simulink model "fft_direct_maptail_test"  (Simulink 7.2)
settings: Solver=VariableStepDiscrete  StartTime=0.0  StopTime=250  RelTol=1e-3
libraries: xbsIndex_r4 x1029, casper_library_misc x88, simulink x2
(part 6 of 9)

== system fft_direct_maptail_test/fft_direct/butterfly1_1/twiddle ==
  a : Inport
  b : Inport  Port=2
  sync : Inport  Port=3
  AddSub : xbsIndex_r4/AddSub  mode=Subtraction  use_carryin=off  use_carryout=off  en=off  latency=add_latency  precision=Full  arith_type=Unsigned  n_bits=16  bin_pt=14  quantization=Truncate  overflow=Wrap  dbl_ovrd=off  use_behavioral_HDL=on  hw_selection=Fabric  pipelined=off  block_type=addsub
  AddSub1 : xbsIndex_r4/AddSub  mode=Addition  use_carryin=off  use_carryout=off  en=off  latency=add_latency  precision=Full  arith_type=Unsigned  n_bits=16  bin_pt=14  quantization=Truncate  overflow=Wrap  dbl_ovrd=off  use_behavioral_HDL=on  hw_selection=Fabric  pipelined=off  block_type=addsub
  c_to_ri1 : casper_library_misc/c_to_ri  SystemSampleTime=-1  n_bits=input_bit_width  bin_pt=input_bit_width-1
      settings: AttributesFormatString=16_15 r/i
  c_to_ri2 : casper_library_misc/c_to_ri  SystemSampleTime=-1  n_bits=coeff_bit_width  bin_pt=coeff_bit_width-2
      settings: AttributesFormatString=16_14 r/i
  c_to_ri3 : casper_library_misc/c_to_ri  SystemSampleTime=-1  n_bits=input_bit_width  bin_pt=input_bit_width-1
      settings: AttributesFormatString=16_15 r/i
  coeff_gen : Subsystem  AncestorBlock=casper_library_ffts_twiddle_coeff_gen/coeff_gen  mask(coeff_gen){Coeffs=getfield( getfield( get_param( gcb,'UserData' ), 'parameters'),'Coeffs'), coeff_bit_width=16, StepPeriod=0, bram_latency=2, coeffs_bram=off}
      mask prompts: Coeffs "Coefficients: (0 to 2^(FFTSize-1)-1)"; coeff_bit_width "Coefficient Bit Width:"; StepPeriod "Step Period: (2^?)"; bram_latency "Latency:"; coeffs_bram "Store coefficients in BRAM"
      mask help: Generates a sequence of complex coefficients
      mask init:
      | coeff_gen_init( gcb, ...
      |     'Coeffs', Coeffs, ...
      |     'coeff_bit_width', coeff_bit_width, ...
      |     'StepPeriod', StepPeriod, ...
      |     'bram_latency', bram_latency, ...
      |     'coeffs_bram', coeffs_bram);
      settings: AttributesFormatString=4 @ (16,14)
      mask CallbackString:
      | Coeffs = eval(get_param(gcb, 'Coeffs'));
      | if( length(Coeffs) == 1 ),
      |     set_param(gcb, 'MaskVisibilities',{'on','on','off','off','off'});
      | else
      |     set_param(gcb, 'MaskVisibilities',{'on','on','on','on','on'});
      | end||||
  convert0 : xbsIndex_r4/Convert  arith_type="Signed  (2's comp)"  n_bits=input_bit_width+4  bin_pt=input_bit_width+1  quantization=Truncate  overflow=Wrap  latency=conv_latency  dbl_ovrd=off  pipeline=on  block_type=convert
      settings: block_version=11.4
  convert1 : xbsIndex_r4/Convert  arith_type="Signed  (2's comp)"  n_bits=input_bit_width+4  bin_pt=input_bit_width+1  quantization=Truncate  overflow=Wrap  latency=conv_latency  dbl_ovrd=off  pipeline=on  block_type=convert
      settings: block_version=11.4
  delay0 : xbsIndex_r4/Delay  en=off  latency=mult_latency + add_latency + bram_latency + conv_latency  dbl_ovrd=off  reg_retiming=off  block_type=delay
      settings: block_version=11.4
  delay1 : xbsIndex_r4/Delay  en=off  latency=bram_latency  dbl_ovrd=off  reg_retiming=on  block_type=delay
      settings: block_version=11.4
  delay2 : xbsIndex_r4/Delay  en=off  latency=mult_latency + add_latency + bram_latency + conv_latency  dbl_ovrd=off  reg_retiming=off  block_type=delay
      settings: block_version=11.4
  mult{,1..3} (4 alike) : xbsIndex_r4/Mult  precision=Full  arith_type="Signed  (2's comp)"  n_bits=16  bin_pt=14  quantization=Truncate  overflow=Wrap  en=off  latency=mult_latency  dbl_ovrd=off  use_behavioral_HDL=on  opt=Speed  use_embedded=off  optimum_pipeline=off  pipeline=on  use_rpm=on  placement_style=Triangular  block_type=mult
      settings: block_version=11.4
  a_re : Outport
  a_im : Outport  Port=2
  bw_re : Outport  Port=3
  bw_im : Outport  Port=4
  sync_out : Outport  Port=5
  wires:
  a/1 -> delay0/1
  delay0/1 -> c_to_ri1/1
  c_to_ri1/1 -> a_re/1
  c_to_ri1/2 -> a_im/1
  sync/1 -> delay2/1, coeff_gen/1(rst)
  delay2/1 -> sync_out/1
  coeff_gen/1(w) -> c_to_ri2/1
  b/1 -> delay1/1
  delay1/1 -> c_to_ri3/1
  c_to_ri3/1 -> mult/1, mult3/1
  c_to_ri2/1 -> mult/2, mult1/2
  c_to_ri3/2 -> mult1/1, mult2/1
  c_to_ri2/2 -> mult2/2, mult3/2
  mult/1 -> AddSub/1
  mult1/1 -> AddSub1/1
  mult2/1 -> AddSub/2
  mult3/1 -> AddSub1/2
  AddSub/1 -> convert0/1
  convert0/1 -> bw_re/1
  AddSub1/1 -> convert1/1
  convert1/1 -> bw_im/1

== system fft_direct_maptail_test/fft_direct/butterfly1_2/convert_of1 ==
  din : Inport  OutDataType=sfix(16)  OutScaling=2^0
  all_0s : xbsIndex_r4/Logical  logical_function=NAND  inputs=4  en=off  latency=latency  precision=Full  arith_type=Unsigned  n_bits=16  bin_pt=0  align_bp=on  dbl_ovrd=off  block_type=logical
  all_1s : xbsIndex_r4/Logical  logical_function=NAND  inputs=4  en=off  latency=latency  precision=Full  arith_type=Unsigned  n_bits=16  bin_pt=0  align_bp=on  dbl_ovrd=off  block_type=logical
  and : xbsIndex_r4/Logical  logical_function=AND  inputs=2  en=off  latency=0  precision=Full  arith_type=Unsigned  n_bits=16  bin_pt=0  align_bp=on  dbl_ovrd=off  block_type=logical
  convert : xbsIndex_r4/Convert  arith_type="Signed  (2's comp)"  n_bits=bit_width_o  bin_pt=binary_point_o  quantization=Truncate  overflow=Wrap  latency=latency  dbl_ovrd=off  pipeline=on  block_type=convert
      settings: block_version=10.1.1
  invert{1..4} (4 alike) : xbsIndex_r4/Inverter  en=off  latency=0  dbl_ovrd=off  block_type=inv
      invert3 settings: block_version=11.4
      invert4 settings: block_version=11.4
  slice1 : xbsIndex_r4/Slice  nbits=1  boolean_output=on  mode=Upper Bit Location + Width  bit1=0  base1=MSB of Input  bit0=0  base0=LSB of Input  dbl_ovrd=off  block_type=slice
      settings: infoedit="Extracts a given range of bits from each input sample and presents it at the output.  The output type is ordinarily unsigned with binary point at zero, but can be Boolean when the slice is one bit wide.<P><P>Hardware notes: In hardware this block costs nothing."  block_version=10.1.1
  slice2 : xbsIndex_r4/Slice  nbits=1  boolean_output=on  mode=Upper Bit Location + Width  bit1=-1  base1=MSB of Input  bit0=0  base0=LSB of Input  dbl_ovrd=off  block_type=slice
      settings: infoedit="Extracts a given range of bits from each input sample and presents it at the output.  The output type is ordinarily unsigned with binary point at zero, but can be Boolean when the slice is one bit wide.<P><P>Hardware notes: In hardware this block costs nothing."  block_version=10.1.1
  slice3 : xbsIndex_r4/Slice  nbits=1  boolean_output=on  mode=Upper Bit Location + Width  bit1=-2  base1=MSB of Input  bit0=0  base0=LSB of Input  dbl_ovrd=off  block_type=slice
  slice4 : xbsIndex_r4/Slice  nbits=1  boolean_output=on  mode=Upper Bit Location + Width  bit1=-3  base1=MSB of Input  bit0=0  base0=LSB of Input  dbl_ovrd=off  block_type=slice
  dout : Outport
  of : Outport  Port=2
  wires:
  din/1 -> convert/1, slice1/1, slice2/1, slice3/1, slice4/1
  convert/1 -> dout/1
  slice1/1 -> all_1s/1, invert1/1
  invert1/1 -> all_0s/1
  slice2/1 -> all_1s/2, invert2/1
  invert2/1 -> all_0s/2
  slice3/1 -> all_1s/3, invert3/1
  invert3/1 -> all_0s/3
  slice4/1 -> all_1s/4, invert4/1
  invert4/1 -> all_0s/4
  all_0s/1 -> and/1
  all_1s/1 -> and/2
  and/1 -> of/1

== system fft_direct_maptail_test/fft_direct/butterfly1_2/convert_of2 ==
  din : Inport  OutDataType=sfix(16)  OutScaling=2^0
  all_0s : xbsIndex_r4/Logical  logical_function=NAND  inputs=4  en=off  latency=latency  precision=Full  arith_type=Unsigned  n_bits=16  bin_pt=0  align_bp=on  dbl_ovrd=off  block_type=logical
  all_1s : xbsIndex_r4/Logical  logical_function=NAND  inputs=4  en=off  latency=latency  precision=Full  arith_type=Unsigned  n_bits=16  bin_pt=0  align_bp=on  dbl_ovrd=off  block_type=logical
  and : xbsIndex_r4/Logical  logical_function=AND  inputs=2  en=off  latency=0  precision=Full  arith_type=Unsigned  n_bits=16  bin_pt=0  align_bp=on  dbl_ovrd=off  block_type=logical
  convert : xbsIndex_r4/Convert  arith_type="Signed  (2's comp)"  n_bits=bit_width_o  bin_pt=binary_point_o  quantization=Truncate  overflow=Wrap  latency=latency  dbl_ovrd=off  pipeline=on  block_type=convert
      settings: block_version=10.1.1
  invert{1..4} (4 alike) : xbsIndex_r4/Inverter  en=off  latency=0  dbl_ovrd=off  block_type=inv
      invert3 settings: block_version=11.4
      invert4 settings: block_version=11.4
  slice1 : xbsIndex_r4/Slice  nbits=1  boolean_output=on  mode=Upper Bit Location + Width  bit1=0  base1=MSB of Input  bit0=0  base0=LSB of Input  dbl_ovrd=off  block_type=slice
      settings: infoedit="Extracts a given range of bits from each input sample and presents it at the output.  The output type is ordinarily unsigned with binary point at zero, but can be Boolean when the slice is one bit wide.<P><P>Hardware notes: In hardware this block costs nothing."  block_version=10.1.1
  slice2 : xbsIndex_r4/Slice  nbits=1  boolean_output=on  mode=Upper Bit Location + Width  bit1=-1  base1=MSB of Input  bit0=0  base0=LSB of Input  dbl_ovrd=off  block_type=slice
      settings: infoedit="Extracts a given range of bits from each input sample and presents it at the output.  The output type is ordinarily unsigned with binary point at zero, but can be Boolean when the slice is one bit wide.<P><P>Hardware notes: In hardware this block costs nothing."  block_version=10.1.1
  slice3 : xbsIndex_r4/Slice  nbits=1  boolean_output=on  mode=Upper Bit Location + Width  bit1=-2  base1=MSB of Input  bit0=0  base0=LSB of Input  dbl_ovrd=off  block_type=slice
  slice4 : xbsIndex_r4/Slice  nbits=1  boolean_output=on  mode=Upper Bit Location + Width  bit1=-3  base1=MSB of Input  bit0=0  base0=LSB of Input  dbl_ovrd=off  block_type=slice
  dout : Outport
  of : Outport  Port=2
  wires:
  din/1 -> convert/1, slice1/1, slice2/1, slice3/1, slice4/1
  convert/1 -> dout/1
  slice1/1 -> all_1s/1, invert1/1
  invert1/1 -> all_0s/1
  slice2/1 -> all_1s/2, invert2/1
  invert2/1 -> all_0s/2
  slice3/1 -> all_1s/3, invert3/1
  invert3/1 -> all_0s/3
  slice4/1 -> all_1s/4, invert4/1
  invert4/1 -> all_0s/4
  all_0s/1 -> and/1
  all_1s/1 -> and/2
  and/1 -> of/1

== system fft_direct_maptail_test/fft_direct/butterfly1_2/convert_of3 ==
  din : Inport  OutDataType=sfix(16)  OutScaling=2^0
  all_0s : xbsIndex_r4/Logical  logical_function=NAND  inputs=4  en=off  latency=latency  precision=Full  arith_type=Unsigned  n_bits=16  bin_pt=0  align_bp=on  dbl_ovrd=off  block_type=logical
  all_1s : xbsIndex_r4/Logical  logical_function=NAND  inputs=4  en=off  latency=latency  precision=Full  arith_type=Unsigned  n_bits=16  bin_pt=0  align_bp=on  dbl_ovrd=off  block_type=logical
  and : xbsIndex_r4/Logical  logical_function=AND  inputs=2  en=off  latency=0  precision=Full  arith_type=Unsigned  n_bits=16  bin_pt=0  align_bp=on  dbl_ovrd=off  block_type=logical
  convert : xbsIndex_r4/Convert  arith_type="Signed  (2's comp)"  n_bits=bit_width_o  bin_pt=binary_point_o  quantization=Truncate  overflow=Wrap  latency=latency  dbl_ovrd=off  pipeline=on  block_type=convert
      settings: block_version=10.1.1
  invert{1..4} (4 alike) : xbsIndex_r4/Inverter  en=off  latency=0  dbl_ovrd=off  block_type=inv
      invert3 settings: block_version=11.4
      invert4 settings: block_version=11.4
  slice1 : xbsIndex_r4/Slice  nbits=1  boolean_output=on  mode=Upper Bit Location + Width  bit1=0  base1=MSB of Input  bit0=0  base0=LSB of Input  dbl_ovrd=off  block_type=slice
      settings: infoedit="Extracts a given range of bits from each input sample and presents it at the output.  The output type is ordinarily unsigned with binary point at zero, but can be Boolean when the slice is one bit wide.<P><P>Hardware notes: In hardware this block costs nothing."  block_version=10.1.1
  slice2 : xbsIndex_r4/Slice  nbits=1  boolean_output=on  mode=Upper Bit Location + Width  bit1=-1  base1=MSB of Input  bit0=0  base0=LSB of Input  dbl_ovrd=off  block_type=slice
      settings: infoedit="Extracts a given range of bits from each input sample and presents it at the output.  The output type is ordinarily unsigned with binary point at zero, but can be Boolean when the slice is one bit wide.<P><P>Hardware notes: In hardware this block costs nothing."  block_version=10.1.1
  slice3 : xbsIndex_r4/Slice  nbits=1  boolean_output=on  mode=Upper Bit Location + Width  bit1=-2  base1=MSB of Input  bit0=0  base0=LSB of Input  dbl_ovrd=off  block_type=slice
  slice4 : xbsIndex_r4/Slice  nbits=1  boolean_output=on  mode=Upper Bit Location + Width  bit1=-3  base1=MSB of Input  bit0=0  base0=LSB of Input  dbl_ovrd=off  block_type=slice
  dout : Outport
  of : Outport  Port=2
  wires:
  din/1 -> convert/1, slice1/1, slice2/1, slice3/1, slice4/1
  convert/1 -> dout/1
  slice1/1 -> all_1s/1, invert1/1
  invert1/1 -> all_0s/1
  slice2/1 -> all_1s/2, invert2/1
  invert2/1 -> all_0s/2
  slice3/1 -> all_1s/3, invert3/1
  invert3/1 -> all_0s/3
  slice4/1 -> all_1s/4, invert4/1
  invert4/1 -> all_0s/4
  all_0s/1 -> and/1
  all_1s/1 -> and/2
  and/1 -> of/1

== system fft_direct_maptail_test/fft_direct/butterfly1_2/convert_of4 ==
  din : Inport  OutDataType=sfix(16)  OutScaling=2^0
  all_0s : xbsIndex_r4/Logical  logical_function=NAND  inputs=4  en=off  latency=latency  precision=Full  arith_type=Unsigned  n_bits=16  bin_pt=0  align_bp=on  dbl_ovrd=off  block_type=logical
  all_1s : xbsIndex_r4/Logical  logical_function=NAND  inputs=4  en=off  latency=latency  precision=Full  arith_type=Unsigned  n_bits=16  bin_pt=0  align_bp=on  dbl_ovrd=off  block_type=logical
  and : xbsIndex_r4/Logical  logical_function=AND  inputs=2  en=off  latency=0  precision=Full  arith_type=Unsigned  n_bits=16  bin_pt=0  align_bp=on  dbl_ovrd=off  block_type=logical
  convert : xbsIndex_r4/Convert  arith_type="Signed  (2's comp)"  n_bits=bit_width_o  bin_pt=binary_point_o  quantization=Truncate  overflow=Wrap  latency=latency  dbl_ovrd=off  pipeline=on  block_type=convert
      settings: block_version=10.1.1
  invert{1..4} (4 alike) : xbsIndex_r4/Inverter  en=off  latency=0  dbl_ovrd=off  block_type=inv
      invert3 settings: block_version=11.4
      invert4 settings: block_version=11.4
  slice1 : xbsIndex_r4/Slice  nbits=1  boolean_output=on  mode=Upper Bit Location + Width  bit1=0  base1=MSB of Input  bit0=0  base0=LSB of Input  dbl_ovrd=off  block_type=slice
      settings: infoedit="Extracts a given range of bits from each input sample and presents it at the output.  The output type is ordinarily unsigned with binary point at zero, but can be Boolean when the slice is one bit wide.<P><P>Hardware notes: In hardware this block costs nothing."  block_version=10.1.1
  slice2 : xbsIndex_r4/Slice  nbits=1  boolean_output=on  mode=Upper Bit Location + Width  bit1=-1  base1=MSB of Input  bit0=0  base0=LSB of Input  dbl_ovrd=off  block_type=slice
      settings: infoedit="Extracts a given range of bits from each input sample and presents it at the output.  The output type is ordinarily unsigned with binary point at zero, but can be Boolean when the slice is one bit wide.<P><P>Hardware notes: In hardware this block costs nothing."  block_version=10.1.1
  slice3 : xbsIndex_r4/Slice  nbits=1  boolean_output=on  mode=Upper Bit Location + Width  bit1=-2  base1=MSB of Input  bit0=0  base0=LSB of Input  dbl_ovrd=off  block_type=slice
  slice4 : xbsIndex_r4/Slice  nbits=1  boolean_output=on  mode=Upper Bit Location + Width  bit1=-3  base1=MSB of Input  bit0=0  base0=LSB of Input  dbl_ovrd=off  block_type=slice
  dout : Outport
  of : Outport  Port=2
  wires:
  din/1 -> convert/1, slice1/1, slice2/1, slice3/1, slice4/1
  convert/1 -> dout/1
  slice1/1 -> all_1s/1, invert1/1
  invert1/1 -> all_0s/1
  slice2/1 -> all_1s/2, invert2/1
  invert2/1 -> all_0s/2
  slice3/1 -> all_1s/3, invert3/1
  invert3/1 -> all_0s/3
  slice4/1 -> all_1s/4, invert4/1
  invert4/1 -> all_0s/4
  all_0s/1 -> and/1
  all_1s/1 -> and/2
  and/1 -> of/1

== system fft_direct_maptail_test/fft_direct/butterfly1_2/twiddle ==
  a : Inport
  b : Inport  Port=2
  sync : Inport  Port=3
  AddSub : xbsIndex_r4/AddSub  mode=Subtraction  use_carryin=off  use_carryout=off  en=off  latency=add_latency  precision=Full  arith_type=Unsigned  n_bits=16  bin_pt=14  quantization=Truncate  overflow=Wrap  dbl_ovrd=off  use_behavioral_HDL=on  hw_selection=Fabric  pipelined=off  block_type=addsub
  AddSub1 : xbsIndex_r4/AddSub  mode=Addition  use_carryin=off  use_carryout=off  en=off  latency=add_latency  precision=Full  arith_type=Unsigned  n_bits=16  bin_pt=14  quantization=Truncate  overflow=Wrap  dbl_ovrd=off  use_behavioral_HDL=on  hw_selection=Fabric  pipelined=off  block_type=addsub
  c_to_ri1 : casper_library_misc/c_to_ri  SystemSampleTime=-1  n_bits=input_bit_width  bin_pt=input_bit_width-1
      settings: AttributesFormatString=16_15 r/i
  c_to_ri2 : casper_library_misc/c_to_ri  SystemSampleTime=-1  n_bits=coeff_bit_width  bin_pt=coeff_bit_width-2
      settings: AttributesFormatString=16_14 r/i
  c_to_ri3 : casper_library_misc/c_to_ri  SystemSampleTime=-1  n_bits=input_bit_width  bin_pt=input_bit_width-1
      settings: AttributesFormatString=16_15 r/i
  coeff_gen : Subsystem  AncestorBlock=casper_library_ffts_twiddle_coeff_gen/coeff_gen  mask(coeff_gen){Coeffs=getfield( getfield( get_param( gcb,'UserData' ), 'parameters'),'Coeffs'), coeff_bit_width=16, StepPeriod=0, bram_latency=2, coeffs_bram=off}
      mask prompts: Coeffs "Coefficients: (0 to 2^(FFTSize-1)-1)"; coeff_bit_width "Coefficient Bit Width:"; StepPeriod "Step Period: (2^?)"; bram_latency "Latency:"; coeffs_bram "Store coefficients in BRAM"
      mask help: Generates a sequence of complex coefficients
      mask init:
      | coeff_gen_init( gcb, ...
      |     'Coeffs', Coeffs, ...
      |     'coeff_bit_width', coeff_bit_width, ...
      |     'StepPeriod', StepPeriod, ...
      |     'bram_latency', bram_latency, ...
      |     'coeffs_bram', coeffs_bram);
      settings: AttributesFormatString=4 @ (16,14)
      mask CallbackString:
      | Coeffs = eval(get_param(gcb, 'Coeffs'));
      | if( length(Coeffs) == 1 ),
      |     set_param(gcb, 'MaskVisibilities',{'on','on','off','off','off'});
      | else
      |     set_param(gcb, 'MaskVisibilities',{'on','on','on','on','on'});
      | end||||
  convert0 : xbsIndex_r4/Convert  arith_type="Signed  (2's comp)"  n_bits=input_bit_width+4  bin_pt=input_bit_width+1  quantization=Truncate  overflow=Wrap  latency=conv_latency  dbl_ovrd=off  pipeline=on  block_type=convert
      settings: block_version=11.4
  convert1 : xbsIndex_r4/Convert  arith_type="Signed  (2's comp)"  n_bits=input_bit_width+4  bin_pt=input_bit_width+1  quantization=Truncate  overflow=Wrap  latency=conv_latency  dbl_ovrd=off  pipeline=on  block_type=convert
      settings: block_version=11.4
  delay0 : xbsIndex_r4/Delay  en=off  latency=mult_latency + add_latency + bram_latency + conv_latency  dbl_ovrd=off  reg_retiming=off  block_type=delay
      settings: block_version=11.4
  delay1 : xbsIndex_r4/Delay  en=off  latency=bram_latency  dbl_ovrd=off  reg_retiming=on  block_type=delay
      settings: block_version=11.4
  delay2 : xbsIndex_r4/Delay  en=off  latency=mult_latency + add_latency + bram_latency + conv_latency  dbl_ovrd=off  reg_retiming=off  block_type=delay
      settings: block_version=11.4
  mult{,1..3} (4 alike) : xbsIndex_r4/Mult  precision=Full  arith_type="Signed  (2's comp)"  n_bits=16  bin_pt=14  quantization=Truncate  overflow=Wrap  en=off  latency=mult_latency  dbl_ovrd=off  use_behavioral_HDL=on  opt=Speed  use_embedded=off  optimum_pipeline=off  pipeline=on  use_rpm=on  placement_style=Triangular  block_type=mult
      settings: block_version=11.4
  a_re : Outport
  a_im : Outport  Port=2
  bw_re : Outport  Port=3
  bw_im : Outport  Port=4
  sync_out : Outport  Port=5
  wires:
  a/1 -> delay0/1
  delay0/1 -> c_to_ri1/1
  c_to_ri1/1 -> a_re/1
  c_to_ri1/2 -> a_im/1
  sync/1 -> delay2/1, coeff_gen/1(rst)
  delay2/1 -> sync_out/1
  coeff_gen/1(w) -> c_to_ri2/1
  b/1 -> delay1/1
  delay1/1 -> c_to_ri3/1
  c_to_ri3/1 -> mult/1, mult3/1
  c_to_ri2/1 -> mult/2, mult1/2
  c_to_ri3/2 -> mult1/1, mult2/1
  c_to_ri2/2 -> mult2/2, mult3/2
  mult/1 -> AddSub/1
  mult1/1 -> AddSub1/1
  mult2/1 -> AddSub/2
  mult3/1 -> AddSub1/2
  AddSub/1 -> convert0/1
  convert0/1 -> bw_re/1
  AddSub1/1 -> convert1/1
  convert1/1 -> bw_im/1

== system fft_direct_maptail_test/fft_direct/butterfly1_3/convert_of1 ==
  din : Inport  OutDataType=sfix(16)  OutScaling=2^0
  all_0s : xbsIndex_r4/Logical  logical_function=NAND  inputs=4  en=off  latency=latency  precision=Full  arith_type=Unsigned  n_bits=16  bin_pt=0  align_bp=on  dbl_ovrd=off  block_type=logical
  all_1s : xbsIndex_r4/Logical  logical_function=NAND  inputs=4  en=off  latency=latency  precision=Full  arith_type=Unsigned  n_bits=16  bin_pt=0  align_bp=on  dbl_ovrd=off  block_type=logical
  and : xbsIndex_r4/Logical  logical_function=AND  inputs=2  en=off  latency=0  precision=Full  arith_type=Unsigned  n_bits=16  bin_pt=0  align_bp=on  dbl_ovrd=off  block_type=logical
  convert : xbsIndex_r4/Convert  arith_type="Signed  (2's comp)"  n_bits=bit_width_o  bin_pt=binary_point_o  quantization=Truncate  overflow=Wrap  latency=latency  dbl_ovrd=off  pipeline=on  block_type=convert
      settings: block_version=10.1.1
  invert{1..4} (4 alike) : xbsIndex_r4/Inverter  en=off  latency=0  dbl_ovrd=off  block_type=inv
      invert3 settings: block_version=11.4
      invert4 settings: block_version=11.4
  slice1 : xbsIndex_r4/Slice  nbits=1  boolean_output=on  mode=Upper Bit Location + Width  bit1=0  base1=MSB of Input  bit0=0  base0=LSB of Input  dbl_ovrd=off  block_type=slice
      settings: infoedit="Extracts a given range of bits from each input sample and presents it at the output.  The output type is ordinarily unsigned with binary point at zero, but can be Boolean when the slice is one bit wide.<P><P>Hardware notes: In hardware this block costs nothing."  block_version=10.1.1
  slice2 : xbsIndex_r4/Slice  nbits=1  boolean_output=on  mode=Upper Bit Location + Width  bit1=-1  base1=MSB of Input  bit0=0  base0=LSB of Input  dbl_ovrd=off  block_type=slice
      settings: infoedit="Extracts a given range of bits from each input sample and presents it at the output.  The output type is ordinarily unsigned with binary point at zero, but can be Boolean when the slice is one bit wide.<P><P>Hardware notes: In hardware this block costs nothing."  block_version=10.1.1
  slice3 : xbsIndex_r4/Slice  nbits=1  boolean_output=on  mode=Upper Bit Location + Width  bit1=-2  base1=MSB of Input  bit0=0  base0=LSB of Input  dbl_ovrd=off  block_type=slice
  slice4 : xbsIndex_r4/Slice  nbits=1  boolean_output=on  mode=Upper Bit Location + Width  bit1=-3  base1=MSB of Input  bit0=0  base0=LSB of Input  dbl_ovrd=off  block_type=slice
  dout : Outport
  of : Outport  Port=2
  wires:
  din/1 -> convert/1, slice1/1, slice2/1, slice3/1, slice4/1
  convert/1 -> dout/1
  slice1/1 -> all_1s/1, invert1/1
  invert1/1 -> all_0s/1
  slice2/1 -> all_1s/2, invert2/1
  invert2/1 -> all_0s/2
  slice3/1 -> all_1s/3, invert3/1
  invert3/1 -> all_0s/3
  slice4/1 -> all_1s/4, invert4/1
  invert4/1 -> all_0s/4
  all_0s/1 -> and/1
  all_1s/1 -> and/2
  and/1 -> of/1

== system fft_direct_maptail_test/fft_direct/butterfly1_3/convert_of2 ==
  din : Inport  OutDataType=sfix(16)  OutScaling=2^0
  all_0s : xbsIndex_r4/Logical  logical_function=NAND  inputs=4  en=off  latency=latency  precision=Full  arith_type=Unsigned  n_bits=16  bin_pt=0  align_bp=on  dbl_ovrd=off  block_type=logical
  all_1s : xbsIndex_r4/Logical  logical_function=NAND  inputs=4  en=off  latency=latency  precision=Full  arith_type=Unsigned  n_bits=16  bin_pt=0  align_bp=on  dbl_ovrd=off  block_type=logical
  and : xbsIndex_r4/Logical  logical_function=AND  inputs=2  en=off  latency=0  precision=Full  arith_type=Unsigned  n_bits=16  bin_pt=0  align_bp=on  dbl_ovrd=off  block_type=logical
  convert : xbsIndex_r4/Convert  arith_type="Signed  (2's comp)"  n_bits=bit_width_o  bin_pt=binary_point_o  quantization=Truncate  overflow=Wrap  latency=latency  dbl_ovrd=off  pipeline=on  block_type=convert
      settings: block_version=10.1.1
  invert{1..4} (4 alike) : xbsIndex_r4/Inverter  en=off  latency=0  dbl_ovrd=off  block_type=inv
      invert3 settings: block_version=11.4
      invert4 settings: block_version=11.4
  slice1 : xbsIndex_r4/Slice  nbits=1  boolean_output=on  mode=Upper Bit Location + Width  bit1=0  base1=MSB of Input  bit0=0  base0=LSB of Input  dbl_ovrd=off  block_type=slice
      settings: infoedit="Extracts a given range of bits from each input sample and presents it at the output.  The output type is ordinarily unsigned with binary point at zero, but can be Boolean when the slice is one bit wide.<P><P>Hardware notes: In hardware this block costs nothing."  block_version=10.1.1
  slice2 : xbsIndex_r4/Slice  nbits=1  boolean_output=on  mode=Upper Bit Location + Width  bit1=-1  base1=MSB of Input  bit0=0  base0=LSB of Input  dbl_ovrd=off  block_type=slice
      settings: infoedit="Extracts a given range of bits from each input sample and presents it at the output.  The output type is ordinarily unsigned with binary point at zero, but can be Boolean when the slice is one bit wide.<P><P>Hardware notes: In hardware this block costs nothing."  block_version=10.1.1
  slice3 : xbsIndex_r4/Slice  nbits=1  boolean_output=on  mode=Upper Bit Location + Width  bit1=-2  base1=MSB of Input  bit0=0  base0=LSB of Input  dbl_ovrd=off  block_type=slice
  slice4 : xbsIndex_r4/Slice  nbits=1  boolean_output=on  mode=Upper Bit Location + Width  bit1=-3  base1=MSB of Input  bit0=0  base0=LSB of Input  dbl_ovrd=off  block_type=slice
  dout : Outport
  of : Outport  Port=2
  wires:
  din/1 -> convert/1, slice1/1, slice2/1, slice3/1, slice4/1
  convert/1 -> dout/1
  slice1/1 -> all_1s/1, invert1/1
  invert1/1 -> all_0s/1
  slice2/1 -> all_1s/2, invert2/1
  invert2/1 -> all_0s/2
  slice3/1 -> all_1s/3, invert3/1
  invert3/1 -> all_0s/3
  slice4/1 -> all_1s/4, invert4/1
  invert4/1 -> all_0s/4
  all_0s/1 -> and/1
  all_1s/1 -> and/2
  and/1 -> of/1

== system fft_direct_maptail_test/fft_direct/butterfly1_3/convert_of3 ==
  din : Inport  OutDataType=sfix(16)  OutScaling=2^0
  all_0s : xbsIndex_r4/Logical  logical_function=NAND  inputs=4  en=off  latency=latency  precision=Full  arith_type=Unsigned  n_bits=16  bin_pt=0  align_bp=on  dbl_ovrd=off  block_type=logical
  all_1s : xbsIndex_r4/Logical  logical_function=NAND  inputs=4  en=off  latency=latency  precision=Full  arith_type=Unsigned  n_bits=16  bin_pt=0  align_bp=on  dbl_ovrd=off  block_type=logical
  and : xbsIndex_r4/Logical  logical_function=AND  inputs=2  en=off  latency=0  precision=Full  arith_type=Unsigned  n_bits=16  bin_pt=0  align_bp=on  dbl_ovrd=off  block_type=logical
  convert : xbsIndex_r4/Convert  arith_type="Signed  (2's comp)"  n_bits=bit_width_o  bin_pt=binary_point_o  quantization=Truncate  overflow=Wrap  latency=latency  dbl_ovrd=off  pipeline=on  block_type=convert
      settings: block_version=10.1.1
  invert{1..4} (4 alike) : xbsIndex_r4/Inverter  en=off  latency=0  dbl_ovrd=off  block_type=inv
      invert3 settings: block_version=11.4
      invert4 settings: block_version=11.4
  slice1 : xbsIndex_r4/Slice  nbits=1  boolean_output=on  mode=Upper Bit Location + Width  bit1=0  base1=MSB of Input  bit0=0  base0=LSB of Input  dbl_ovrd=off  block_type=slice
      settings: infoedit="Extracts a given range of bits from each input sample and presents it at the output.  The output type is ordinarily unsigned with binary point at zero, but can be Boolean when the slice is one bit wide.<P><P>Hardware notes: In hardware this block costs nothing."  block_version=10.1.1
  slice2 : xbsIndex_r4/Slice  nbits=1  boolean_output=on  mode=Upper Bit Location + Width  bit1=-1  base1=MSB of Input  bit0=0  base0=LSB of Input  dbl_ovrd=off  block_type=slice
      settings: infoedit="Extracts a given range of bits from each input sample and presents it at the output.  The output type is ordinarily unsigned with binary point at zero, but can be Boolean when the slice is one bit wide.<P><P>Hardware notes: In hardware this block costs nothing."  block_version=10.1.1
  slice3 : xbsIndex_r4/Slice  nbits=1  boolean_output=on  mode=Upper Bit Location + Width  bit1=-2  base1=MSB of Input  bit0=0  base0=LSB of Input  dbl_ovrd=off  block_type=slice
  slice4 : xbsIndex_r4/Slice  nbits=1  boolean_output=on  mode=Upper Bit Location + Width  bit1=-3  base1=MSB of Input  bit0=0  base0=LSB of Input  dbl_ovrd=off  block_type=slice
  dout : Outport
  of : Outport  Port=2
  wires:
  din/1 -> convert/1, slice1/1, slice2/1, slice3/1, slice4/1
  convert/1 -> dout/1
  slice1/1 -> all_1s/1, invert1/1
  invert1/1 -> all_0s/1
  slice2/1 -> all_1s/2, invert2/1
  invert2/1 -> all_0s/2
  slice3/1 -> all_1s/3, invert3/1
  invert3/1 -> all_0s/3
  slice4/1 -> all_1s/4, invert4/1
  invert4/1 -> all_0s/4
  all_0s/1 -> and/1
  all_1s/1 -> and/2
  and/1 -> of/1

== system fft_direct_maptail_test/fft_direct/butterfly1_3/convert_of4 ==
  din : Inport  OutDataType=sfix(16)  OutScaling=2^0
  all_0s : xbsIndex_r4/Logical  logical_function=NAND  inputs=4  en=off  latency=latency  precision=Full  arith_type=Unsigned  n_bits=16  bin_pt=0  align_bp=on  dbl_ovrd=off  block_type=logical
  all_1s : xbsIndex_r4/Logical  logical_function=NAND  inputs=4  en=off  latency=latency  precision=Full  arith_type=Unsigned  n_bits=16  bin_pt=0  align_bp=on  dbl_ovrd=off  block_type=logical
  and : xbsIndex_r4/Logical  logical_function=AND  inputs=2  en=off  latency=0  precision=Full  arith_type=Unsigned  n_bits=16  bin_pt=0  align_bp=on  dbl_ovrd=off  block_type=logical
  convert : xbsIndex_r4/Convert  arith_type="Signed  (2's comp)"  n_bits=bit_width_o  bin_pt=binary_point_o  quantization=Truncate  overflow=Wrap  latency=latency  dbl_ovrd=off  pipeline=on  block_type=convert
      settings: block_version=10.1.1
  invert{1..4} (4 alike) : xbsIndex_r4/Inverter  en=off  latency=0  dbl_ovrd=off  block_type=inv
      invert3 settings: block_version=11.4
      invert4 settings: block_version=11.4
  slice1 : xbsIndex_r4/Slice  nbits=1  boolean_output=on  mode=Upper Bit Location + Width  bit1=0  base1=MSB of Input  bit0=0  base0=LSB of Input  dbl_ovrd=off  block_type=slice
      settings: infoedit="Extracts a given range of bits from each input sample and presents it at the output.  The output type is ordinarily unsigned with binary point at zero, but can be Boolean when the slice is one bit wide.<P><P>Hardware notes: In hardware this block costs nothing."  block_version=10.1.1
  slice2 : xbsIndex_r4/Slice  nbits=1  boolean_output=on  mode=Upper Bit Location + Width  bit1=-1  base1=MSB of Input  bit0=0  base0=LSB of Input  dbl_ovrd=off  block_type=slice
      settings: infoedit="Extracts a given range of bits from each input sample and presents it at the output.  The output type is ordinarily unsigned with binary point at zero, but can be Boolean when the slice is one bit wide.<P><P>Hardware notes: In hardware this block costs nothing."  block_version=10.1.1
  slice3 : xbsIndex_r4/Slice  nbits=1  boolean_output=on  mode=Upper Bit Location + Width  bit1=-2  base1=MSB of Input  bit0=0  base0=LSB of Input  dbl_ovrd=off  block_type=slice
  slice4 : xbsIndex_r4/Slice  nbits=1  boolean_output=on  mode=Upper Bit Location + Width  bit1=-3  base1=MSB of Input  bit0=0  base0=LSB of Input  dbl_ovrd=off  block_type=slice
  dout : Outport
  of : Outport  Port=2
  wires:
  din/1 -> convert/1, slice1/1, slice2/1, slice3/1, slice4/1
  convert/1 -> dout/1
  slice1/1 -> all_1s/1, invert1/1
  invert1/1 -> all_0s/1
  slice2/1 -> all_1s/2, invert2/1
  invert2/1 -> all_0s/2
  slice3/1 -> all_1s/3, invert3/1
  invert3/1 -> all_0s/3
  slice4/1 -> all_1s/4, invert4/1
  invert4/1 -> all_0s/4
  all_0s/1 -> and/1
  all_1s/1 -> and/2
  and/1 -> of/1

== system fft_direct_maptail_test/fft_direct/butterfly1_3/twiddle ==
  a : Inport
  b : Inport  Port=2
  sync : Inport  Port=3
  AddSub : xbsIndex_r4/AddSub  mode=Subtraction  use_carryin=off  use_carryout=off  en=off  latency=add_latency  precision=Full  arith_type=Unsigned  n_bits=16  bin_pt=14  quantization=Truncate  overflow=Wrap  dbl_ovrd=off  use_behavioral_HDL=on  hw_selection=Fabric  pipelined=off  block_type=addsub
  AddSub1 : xbsIndex_r4/AddSub  mode=Addition  use_carryin=off  use_carryout=off  en=off  latency=add_latency  precision=Full  arith_type=Unsigned  n_bits=16  bin_pt=14  quantization=Truncate  overflow=Wrap  dbl_ovrd=off  use_behavioral_HDL=on  hw_selection=Fabric  pipelined=off  block_type=addsub
  c_to_ri1 : casper_library_misc/c_to_ri  SystemSampleTime=-1  n_bits=input_bit_width  bin_pt=input_bit_width-1
      settings: AttributesFormatString=16_15 r/i
  c_to_ri2 : casper_library_misc/c_to_ri  SystemSampleTime=-1  n_bits=coeff_bit_width  bin_pt=coeff_bit_width-2
      settings: AttributesFormatString=16_14 r/i
  c_to_ri3 : casper_library_misc/c_to_ri  SystemSampleTime=-1  n_bits=input_bit_width  bin_pt=input_bit_width-1
      settings: AttributesFormatString=16_15 r/i
  coeff_gen : Subsystem  AncestorBlock=casper_library_ffts_twiddle_coeff_gen/coeff_gen  mask(coeff_gen){Coeffs=getfield( getfield( get_param( gcb,'UserData' ), 'parameters'),'Coeffs'), coeff_bit_width=16, StepPeriod=0, bram_latency=2, coeffs_bram=off}
      mask prompts: Coeffs "Coefficients: (0 to 2^(FFTSize-1)-1)"; coeff_bit_width "Coefficient Bit Width:"; StepPeriod "Step Period: (2^?)"; bram_latency "Latency:"; coeffs_bram "Store coefficients in BRAM"
      mask help: Generates a sequence of complex coefficients
      mask init:
      | coeff_gen_init( gcb, ...
      |     'Coeffs', Coeffs, ...
      |     'coeff_bit_width', coeff_bit_width, ...
      |     'StepPeriod', StepPeriod, ...
      |     'bram_latency', bram_latency, ...
      |     'coeffs_bram', coeffs_bram);
      settings: AttributesFormatString=4 @ (16,14)
      mask CallbackString:
      | Coeffs = eval(get_param(gcb, 'Coeffs'));
      | if( length(Coeffs) == 1 ),
      |     set_param(gcb, 'MaskVisibilities',{'on','on','off','off','off'});
      | else
      |     set_param(gcb, 'MaskVisibilities',{'on','on','on','on','on'});
      | end||||
  convert0 : xbsIndex_r4/Convert  arith_type="Signed  (2's comp)"  n_bits=input_bit_width+4  bin_pt=input_bit_width+1  quantization=Truncate  overflow=Wrap  latency=conv_latency  dbl_ovrd=off  pipeline=on  block_type=convert
      settings: block_version=11.4
  convert1 : xbsIndex_r4/Convert  arith_type="Signed  (2's comp)"  n_bits=input_bit_width+4  bin_pt=input_bit_width+1  quantization=Truncate  overflow=Wrap  latency=conv_latency  dbl_ovrd=off  pipeline=on  block_type=convert
      settings: block_version=11.4
  delay0 : xbsIndex_r4/Delay  en=off  latency=mult_latency + add_latency + bram_latency + conv_latency  dbl_ovrd=off  reg_retiming=off  block_type=delay
      settings: block_version=11.4
  delay1 : xbsIndex_r4/Delay  en=off  latency=bram_latency  dbl_ovrd=off  reg_retiming=on  block_type=delay
      settings: block_version=11.4
  delay2 : xbsIndex_r4/Delay  en=off  latency=mult_latency + add_latency + bram_latency + conv_latency  dbl_ovrd=off  reg_retiming=off  block_type=delay
      settings: block_version=11.4
  mult{,1..3} (4 alike) : xbsIndex_r4/Mult  precision=Full  arith_type="Signed  (2's comp)"  n_bits=16  bin_pt=14  quantization=Truncate  overflow=Wrap  en=off  latency=mult_latency  dbl_ovrd=off  use_behavioral_HDL=on  opt=Speed  use_embedded=off  optimum_pipeline=off  pipeline=on  use_rpm=on  placement_style=Triangular  block_type=mult
      settings: block_version=11.4
  a_re : Outport
  a_im : Outport  Port=2
  bw_re : Outport  Port=3
  bw_im : Outport  Port=4
  sync_out : Outport  Port=5
  wires:
  a/1 -> delay0/1
  delay0/1 -> c_to_ri1/1
  c_to_ri1/1 -> a_re/1
  c_to_ri1/2 -> a_im/1
  sync/1 -> delay2/1, coeff_gen/1(rst)
  delay2/1 -> sync_out/1
  coeff_gen/1(w) -> c_to_ri2/1
  b/1 -> delay1/1
  delay1/1 -> c_to_ri3/1
  c_to_ri3/1 -> mult/1, mult3/1
  c_to_ri2/1 -> mult/2, mult1/2
  c_to_ri3/2 -> mult1/1, mult2/1
  c_to_ri2/2 -> mult2/2, mult3/2
  mult/1 -> AddSub/1
  mult1/1 -> AddSub1/1
  mult2/1 -> AddSub/2
  mult3/1 -> AddSub1/2
  AddSub/1 -> convert0/1
  convert0/1 -> bw_re/1
  AddSub1/1 -> convert1/1
  convert1/1 -> bw_im/1

== system fft_direct_maptail_test/fft_direct/butterfly2_0/convert_of1 ==
  din : Inport  OutDataType=sfix(16)  OutScaling=2^0
  all_0s : xbsIndex_r4/Logical  logical_function=NAND  inputs=4  en=off  latency=latency  precision=Full  arith_type=Unsigned  n_bits=16  bin_pt=0  align_bp=on  dbl_ovrd=off  block_type=logical
  all_1s : xbsIndex_r4/Logical  logical_function=NAND  inputs=4  en=off  latency=latency  precision=Full  arith_type=Unsigned  n_bits=16  bin_pt=0  align_bp=on  dbl_ovrd=off  block_type=logical
  and : xbsIndex_r4/Logical  logical_function=AND  inputs=2  en=off  latency=0  precision=Full  arith_type=Unsigned  n_bits=16  bin_pt=0  align_bp=on  dbl_ovrd=off  block_type=logical
  convert : xbsIndex_r4/Convert  arith_type="Signed  (2's comp)"  n_bits=bit_width_o  bin_pt=binary_point_o  quantization=Truncate  overflow=Wrap  latency=latency  dbl_ovrd=off  pipeline=on  block_type=convert
      settings: block_version=10.1.1
  invert{1..4} (4 alike) : xbsIndex_r4/Inverter  en=off  latency=0  dbl_ovrd=off  block_type=inv
      invert3 settings: block_version=11.4
      invert4 settings: block_version=11.4
  slice1 : xbsIndex_r4/Slice  nbits=1  boolean_output=on  mode=Upper Bit Location + Width  bit1=0  base1=MSB of Input  bit0=0  base0=LSB of Input  dbl_ovrd=off  block_type=slice
      settings: infoedit="Extracts a given range of bits from each input sample and presents it at the output.  The output type is ordinarily unsigned with binary point at zero, but can be Boolean when the slice is one bit wide.<P><P>Hardware notes: In hardware this block costs nothing."  block_version=10.1.1
  slice2 : xbsIndex_r4/Slice  nbits=1  boolean_output=on  mode=Upper Bit Location + Width  bit1=-1  base1=MSB of Input  bit0=0  base0=LSB of Input  dbl_ovrd=off  block_type=slice
      settings: infoedit="Extracts a given range of bits from each input sample and presents it at the output.  The output type is ordinarily unsigned with binary point at zero, but can be Boolean when the slice is one bit wide.<P><P>Hardware notes: In hardware this block costs nothing."  block_version=10.1.1
  slice3 : xbsIndex_r4/Slice  nbits=1  boolean_output=on  mode=Upper Bit Location + Width  bit1=-2  base1=MSB of Input  bit0=0  base0=LSB of Input  dbl_ovrd=off  block_type=slice
  slice4 : xbsIndex_r4/Slice  nbits=1  boolean_output=on  mode=Upper Bit Location + Width  bit1=-3  base1=MSB of Input  bit0=0  base0=LSB of Input  dbl_ovrd=off  block_type=slice
  dout : Outport
  of : Outport  Port=2
  wires:
  din/1 -> convert/1, slice1/1, slice2/1, slice3/1, slice4/1
  convert/1 -> dout/1
  slice1/1 -> all_1s/1, invert1/1
  invert1/1 -> all_0s/1
  slice2/1 -> all_1s/2, invert2/1
  invert2/1 -> all_0s/2
  slice3/1 -> all_1s/3, invert3/1
  invert3/1 -> all_0s/3
  slice4/1 -> all_1s/4, invert4/1
  invert4/1 -> all_0s/4
  all_0s/1 -> and/1
  all_1s/1 -> and/2
  and/1 -> of/1

== system fft_direct_maptail_test/fft_direct/butterfly2_0/convert_of2 ==
  din : Inport  OutDataType=sfix(16)  OutScaling=2^0
  all_0s : xbsIndex_r4/Logical  logical_function=NAND  inputs=4  en=off  latency=latency  precision=Full  arith_type=Unsigned  n_bits=16  bin_pt=0  align_bp=on  dbl_ovrd=off  block_type=logical
  all_1s : xbsIndex_r4/Logical  logical_function=NAND  inputs=4  en=off  latency=latency  precision=Full  arith_type=Unsigned  n_bits=16  bin_pt=0  align_bp=on  dbl_ovrd=off  block_type=logical
  and : xbsIndex_r4/Logical  logical_function=AND  inputs=2  en=off  latency=0  precision=Full  arith_type=Unsigned  n_bits=16  bin_pt=0  align_bp=on  dbl_ovrd=off  block_type=logical
  convert : xbsIndex_r4/Convert  arith_type="Signed  (2's comp)"  n_bits=bit_width_o  bin_pt=binary_point_o  quantization=Truncate  overflow=Wrap  latency=latency  dbl_ovrd=off  pipeline=on  block_type=convert
      settings: block_version=10.1.1
  invert{1..4} (4 alike) : xbsIndex_r4/Inverter  en=off  latency=0  dbl_ovrd=off  block_type=inv
      invert3 settings: block_version=11.4
      invert4 settings: block_version=11.4
  slice1 : xbsIndex_r4/Slice  nbits=1  boolean_output=on  mode=Upper Bit Location + Width  bit1=0  base1=MSB of Input  bit0=0  base0=LSB of Input  dbl_ovrd=off  block_type=slice
      settings: infoedit="Extracts a given range of bits from each input sample and presents it at the output.  The output type is ordinarily unsigned with binary point at zero, but can be Boolean when the slice is one bit wide.<P><P>Hardware notes: In hardware this block costs nothing."  block_version=10.1.1
  slice2 : xbsIndex_r4/Slice  nbits=1  boolean_output=on  mode=Upper Bit Location + Width  bit1=-1  base1=MSB of Input  bit0=0  base0=LSB of Input  dbl_ovrd=off  block_type=slice
      settings: infoedit="Extracts a given range of bits from each input sample and presents it at the output.  The output type is ordinarily unsigned with binary point at zero, but can be Boolean when the slice is one bit wide.<P><P>Hardware notes: In hardware this block costs nothing."  block_version=10.1.1
  slice3 : xbsIndex_r4/Slice  nbits=1  boolean_output=on  mode=Upper Bit Location + Width  bit1=-2  base1=MSB of Input  bit0=0  base0=LSB of Input  dbl_ovrd=off  block_type=slice
  slice4 : xbsIndex_r4/Slice  nbits=1  boolean_output=on  mode=Upper Bit Location + Width  bit1=-3  base1=MSB of Input  bit0=0  base0=LSB of Input  dbl_ovrd=off  block_type=slice
  dout : Outport
  of : Outport  Port=2
  wires:
  din/1 -> convert/1, slice1/1, slice2/1, slice3/1, slice4/1
  convert/1 -> dout/1
  slice1/1 -> all_1s/1, invert1/1
  invert1/1 -> all_0s/1
  slice2/1 -> all_1s/2, invert2/1
  invert2/1 -> all_0s/2
  slice3/1 -> all_1s/3, invert3/1
  invert3/1 -> all_0s/3
  slice4/1 -> all_1s/4, invert4/1
  invert4/1 -> all_0s/4
  all_0s/1 -> and/1
  all_1s/1 -> and/2
  and/1 -> of/1

== system fft_direct_maptail_test/fft_direct/butterfly2_0/convert_of3 ==
  din : Inport  OutDataType=sfix(16)  OutScaling=2^0
  all_0s : xbsIndex_r4/Logical  logical_function=NAND  inputs=4  en=off  latency=latency  precision=Full  arith_type=Unsigned  n_bits=16  bin_pt=0  align_bp=on  dbl_ovrd=off  block_type=logical
  all_1s : xbsIndex_r4/Logical  logical_function=NAND  inputs=4  en=off  latency=latency  precision=Full  arith_type=Unsigned  n_bits=16  bin_pt=0  align_bp=on  dbl_ovrd=off  block_type=logical
  and : xbsIndex_r4/Logical  logical_function=AND  inputs=2  en=off  latency=0  precision=Full  arith_type=Unsigned  n_bits=16  bin_pt=0  align_bp=on  dbl_ovrd=off  block_type=logical
  convert : xbsIndex_r4/Convert  arith_type="Signed  (2's comp)"  n_bits=bit_width_o  bin_pt=binary_point_o  quantization=Truncate  overflow=Wrap  latency=latency  dbl_ovrd=off  pipeline=on  block_type=convert
      settings: block_version=10.1.1
  invert{1..4} (4 alike) : xbsIndex_r4/Inverter  en=off  latency=0  dbl_ovrd=off  block_type=inv
      invert3 settings: block_version=11.4
      invert4 settings: block_version=11.4
  slice1 : xbsIndex_r4/Slice  nbits=1  boolean_output=on  mode=Upper Bit Location + Width  bit1=0  base1=MSB of Input  bit0=0  base0=LSB of Input  dbl_ovrd=off  block_type=slice
      settings: infoedit="Extracts a given range of bits from each input sample and presents it at the output.  The output type is ordinarily unsigned with binary point at zero, but can be Boolean when the slice is one bit wide.<P><P>Hardware notes: In hardware this block costs nothing."  block_version=10.1.1
  slice2 : xbsIndex_r4/Slice  nbits=1  boolean_output=on  mode=Upper Bit Location + Width  bit1=-1  base1=MSB of Input  bit0=0  base0=LSB of Input  dbl_ovrd=off  block_type=slice
      settings: infoedit="Extracts a given range of bits from each input sample and presents it at the output.  The output type is ordinarily unsigned with binary point at zero, but can be Boolean when the slice is one bit wide.<P><P>Hardware notes: In hardware this block costs nothing."  block_version=10.1.1
  slice3 : xbsIndex_r4/Slice  nbits=1  boolean_output=on  mode=Upper Bit Location + Width  bit1=-2  base1=MSB of Input  bit0=0  base0=LSB of Input  dbl_ovrd=off  block_type=slice
  slice4 : xbsIndex_r4/Slice  nbits=1  boolean_output=on  mode=Upper Bit Location + Width  bit1=-3  base1=MSB of Input  bit0=0  base0=LSB of Input  dbl_ovrd=off  block_type=slice
  dout : Outport
  of : Outport  Port=2
  wires:
  din/1 -> convert/1, slice1/1, slice2/1, slice3/1, slice4/1
  convert/1 -> dout/1
  slice1/1 -> all_1s/1, invert1/1
  invert1/1 -> all_0s/1
  slice2/1 -> all_1s/2, invert2/1
  invert2/1 -> all_0s/2
  slice3/1 -> all_1s/3, invert3/1
  invert3/1 -> all_0s/3
  slice4/1 -> all_1s/4, invert4/1
  invert4/1 -> all_0s/4
  all_0s/1 -> and/1
  all_1s/1 -> and/2
  and/1 -> of/1

== system fft_direct_maptail_test/fft_direct/butterfly2_0/convert_of4 ==
  din : Inport  OutDataType=sfix(16)  OutScaling=2^0
  all_0s : xbsIndex_r4/Logical  logical_function=NAND  inputs=4  en=off  latency=latency  precision=Full  arith_type=Unsigned  n_bits=16  bin_pt=0  align_bp=on  dbl_ovrd=off  block_type=logical
  all_1s : xbsIndex_r4/Logical  logical_function=NAND  inputs=4  en=off  latency=latency  precision=Full  arith_type=Unsigned  n_bits=16  bin_pt=0  align_bp=on  dbl_ovrd=off  block_type=logical
  and : xbsIndex_r4/Logical  logical_function=AND  inputs=2  en=off  latency=0  precision=Full  arith_type=Unsigned  n_bits=16  bin_pt=0  align_bp=on  dbl_ovrd=off  block_type=logical
  convert : xbsIndex_r4/Convert  arith_type="Signed  (2's comp)"  n_bits=bit_width_o  bin_pt=binary_point_o  quantization=Truncate  overflow=Wrap  latency=latency  dbl_ovrd=off  pipeline=on  block_type=convert
      settings: block_version=10.1.1
  invert{1..4} (4 alike) : xbsIndex_r4/Inverter  en=off  latency=0  dbl_ovrd=off  block_type=inv
      invert3 settings: block_version=11.4
      invert4 settings: block_version=11.4
  slice1 : xbsIndex_r4/Slice  nbits=1  boolean_output=on  mode=Upper Bit Location + Width  bit1=0  base1=MSB of Input  bit0=0  base0=LSB of Input  dbl_ovrd=off  block_type=slice
      settings: infoedit="Extracts a given range of bits from each input sample and presents it at the output.  The output type is ordinarily unsigned with binary point at zero, but can be Boolean when the slice is one bit wide.<P><P>Hardware notes: In hardware this block costs nothing."  block_version=10.1.1
  slice2 : xbsIndex_r4/Slice  nbits=1  boolean_output=on  mode=Upper Bit Location + Width  bit1=-1  base1=MSB of Input  bit0=0  base0=LSB of Input  dbl_ovrd=off  block_type=slice
      settings: infoedit="Extracts a given range of bits from each input sample and presents it at the output.  The output type is ordinarily unsigned with binary point at zero, but can be Boolean when the slice is one bit wide.<P><P>Hardware notes: In hardware this block costs nothing."  block_version=10.1.1
  slice3 : xbsIndex_r4/Slice  nbits=1  boolean_output=on  mode=Upper Bit Location + Width  bit1=-2  base1=MSB of Input  bit0=0  base0=LSB of Input  dbl_ovrd=off  block_type=slice
  slice4 : xbsIndex_r4/Slice  nbits=1  boolean_output=on  mode=Upper Bit Location + Width  bit1=-3  base1=MSB of Input  bit0=0  base0=LSB of Input  dbl_ovrd=off  block_type=slice
  dout : Outport
  of : Outport  Port=2
  wires:
  din/1 -> convert/1, slice1/1, slice2/1, slice3/1, slice4/1
  convert/1 -> dout/1
  slice1/1 -> all_1s/1, invert1/1
  invert1/1 -> all_0s/1
  slice2/1 -> all_1s/2, invert2/1
  invert2/1 -> all_0s/2
  slice3/1 -> all_1s/3, invert3/1
  invert3/1 -> all_0s/3
  slice4/1 -> all_1s/4, invert4/1
  invert4/1 -> all_0s/4
  all_0s/1 -> and/1
  all_1s/1 -> and/2
  and/1 -> of/1
